simulink model "t_drone_interp"  (R2025b)
settings: Solver=VariableStepAuto  StartTime=0.0  StopTime=timespot_spl(end)+4  MaxStep=0.01  RelTol=1e-3
StopFcn:
  | figure(77)
  | plot3(out.xyz.Data(:,1),out.xyz.Data(:,2),out.xyz.Data(:,3),'DisplayName','Simulink Interpolation');
  | hold on
  | plot3(out.xyzML.Data(:,1),out.xyzML.Data(:,2),out.xyzML.Data(:,3),'DisplayName','MATLAB Interpolation');
  | hold off
  | axis equal
  | ah = gca;
  | ah.Clipping = 'off';
  | box on
  | grid on
  | legend('Location','Best')
  | title('Show Interpolated Path');
undefined symbols (not defined in the file): spline_data, timespot_spl
Description:
  | Copyright 2022-2025 The MathWorks, Inc.
settings Model: Creator=smiller  LastModifiedBy=smiller
settings OptimizationCC: ReuseModelBlockBuffer=off
settings DebuggingCC: UnconnectedInputMsg=warning  UnconnectedOutputMsg=warning  UnconnectedLineMsg=warning
settings ModelReferenceCC: EnableRefExpFcnMdlSchedulingChecks=on
settings RTWCC: GPUComputeCapability=3.5  DLArmComputeVersion=19.05

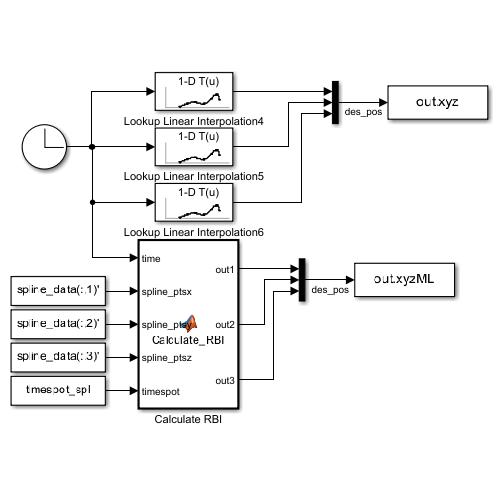
[thumbnail: Simulink's stored preview of the top-level diagram]
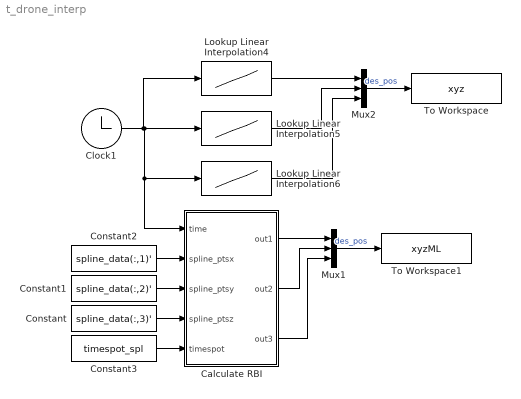
== system t_drone_interp ==
  Calculate RBI : MATLAB Function  TreatAsAtomicUnit=on
  Clock1 : Clock
  Constant : Constant  Value=spline_data(:,3)'
  Constant1 : Constant  Value=spline_data(:,2)'
  Constant2 : Constant  Value=spline_data(:,1)'
  Constant3 : Constant  Value=timespot_spl
  Lookup Linear Interpolation4 : Lookup_n-D  NumberOfTableDimensions=1  BreakpointsForDimension1=timespot_spl  Table=spline_data(:,1)  InterpMethod=Cubic spline  ExtrapMethod=Clip  InternalRulePriority=Speed  RndMeth=Simplest
  Lookup Linear Interpolation5 : Lookup_n-D  NumberOfTableDimensions=1  BreakpointsForDimension1=timespot_spl  Table=spline_data(:,2)  InterpMethod=Cubic spline  ExtrapMethod=Clip  InternalRulePriority=Speed  RndMeth=Simplest
  Lookup Linear Interpolation6 : Lookup_n-D  NumberOfTableDimensions=1  BreakpointsForDimension1=timespot_spl  Table=spline_data(:,3)  InterpMethod=Cubic spline  ExtrapMethod=Clip  InternalRulePriority=Speed  RndMeth=Simplest
  Mux1 : Mux  Inputs=3
  Mux2 : Mux  Inputs=3
  To Workspace : ToWorkspace  VariableName=xyz  SaveFormat=Timeseries  SampleTime=-1
  To Workspace1 : ToWorkspace  VariableName=xyzML  SaveFormat=Timeseries  SampleTime=-1
  wires:
  Clock1/1 -> Lookup Linear Interpolation4/1, Lookup Linear Interpolation5/1, Calculate RBI/1(time), Lookup Linear Interpolation6/1
  Lookup Linear Interpolation4/1 -> Mux2/1
  Lookup Linear Interpolation6/1 -> Mux2/3
  Lookup Linear Interpolation5/1 -> Mux2/2
  Mux2/1 -> To Workspace/1  "des_pos"
  Constant/1 -> Calculate RBI/4(spline_ptsz)
  Constant1/1 -> Calculate RBI/3(spline_ptsy)
  Constant2/1 -> Calculate RBI/2(spline_ptsx)
  Constant3/1 -> Calculate RBI/5(timespot)
  Mux1/1 -> To Workspace1/1  "des_pos"
  Calculate RBI/1(out1) -> Mux1/1
  Calculate RBI/2(out2) -> Mux1/2
  Calculate RBI/3(out3) -> Mux1/3

== matlab function t_drone_interp/Calculate RBI ==
  data: out1 output; time input; spline_ptsx input; spline_ptsy input; spline_ptsz input; timespot input; out2 output; out3 output
function [out1, out2, out3]  = Calculate_RBI(time, spline_ptsx, spline_ptsy, spline_ptsz, timespot)

out1 = interp1(timespot,spline_ptsx,time,'cubic');
out2 = interp1(timespot,spline_ptsy,time,'cubic');
out3 = interp1(timespot,spline_ptsz,time,'cubic');
